simulink model "FMT_MILSIM"  (R2026b)
settings: Solver=FixedStepDiscrete  StopTime=26  FixedStep=0.0005
undefined symbols (not defined in the file): fmt_flight_nav_width, SensorModelParameters, SensorParameters, SensorTimingParameters
settings Model: DataDictionary=Flight_Parameters.sldd  Creator=26718  LastModifiedBy=26718
settings DataIOCC: ExternalInput=fmt_default_input('FMT_MILSIM')  LoadExternalInput=on
settings DebuggingCC: AlgebraicLoopMsg=error

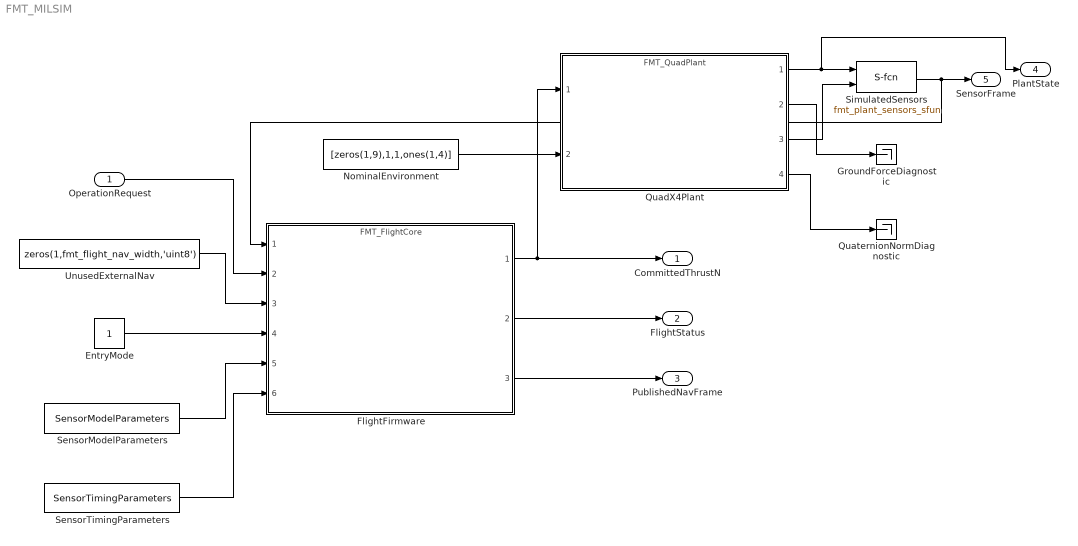
== system FMT_MILSIM ==
  OperationRequest : Inport  OutDataTypeStr=double  PortDimensions=2  SampleTime=0.0005  Interpolate=off
  EntryMode : Constant
  FlightFirmware : ModelReference  ModelNameDialog=FMT_FlightCore  SimulationMode=Normal  ModelReferenceVersion=1.1
  GroundForceDiagnostic : Terminator
  NominalEnvironment : Constant  Value=[zeros(1,9),1,1,ones(1,4)]
  QuadX4Plant : ModelReference  ModelNameDialog=FMT_QuadPlant  SimulationMode=Normal  ModelReferenceVersion=1.1
  QuaternionNormDiagnostic : Terminator
  SensorModelParameters : Constant  Value=SensorModelParameters
  SensorTimingParameters : Constant  Value=SensorTimingParameters
  SimulatedSensors : S-Function  FunctionName=fmt_plant_sensors_sfun  Parameters=SensorParameters,SensorModelParameters,SensorTimingParameters  SFunctionDeploymentMode=off  EnableBusSupport=off
  UnusedExternalNav : Constant  Value=zeros(1,fmt_flight_nav_width,'uint8')  OutDataTypeStr=uint8
  CommittedThrustN : Outport
  FlightStatus : Outport  Port=2
  PublishedNavFrame : Outport  Port=3
  PlantState : Outport  Port=4
  SensorFrame : Outport  Port=5
  wires:
  SensorTimingParameters/1 -> FlightFirmware/6
  SensorModelParameters/1 -> FlightFirmware/5
  OperationRequest/1 -> FlightFirmware/2
  UnusedExternalNav/1 -> FlightFirmware/3
  QuadX4Plant/4 -> QuaternionNormDiagnostic/1
  QuadX4Plant/2 -> GroundForceDiagnostic/1
  SimulatedSensors/1 -> SensorFrame/1, FlightFirmware/1
  QuadX4Plant/3 -> SimulatedSensors/2
  QuadX4Plant/1 -> SimulatedSensors/1, PlantState/1
  NominalEnvironment/1 -> QuadX4Plant/2
  FlightFirmware/3 -> PublishedNavFrame/1
  FlightFirmware/2 -> FlightStatus/1
  FlightFirmware/1 -> CommittedThrustN/1, QuadX4Plant/1
  EntryMode/1 -> FlightFirmware/4
